simulink model "Cubli_2DOFv2"  (R2024b)
settings: Solver=FixedStepAuto  StartTime=0.0  StopTime=30  FixedStep=0.001  RelTol=1e-3  AbsTol=1e-3  EnableMultiTasking=on
values from neighbouring files (symbols this model uses):
  Km = 24.7*10^-3    (= 0.0247)    [cubli_2DOF_LQR.m]
  rad2rpm = 60/(2*pi)    (= 9.54929658551)    [cubli_2DOF_LQR.m]
  switch_time = 10    [cubli_2DOF_LQR.m]
undefined symbols (not defined in the file or in its folder): K, X, Y, Z
libraries: sm_lib x76, nesl_utility x8, simulink_extras x1
(part 2 of 3)

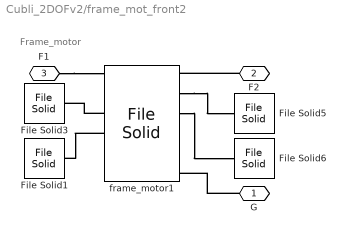
== system Cubli_2DOFv2/frame_mot_front2 ==
  note: Frame_motor
  File Solid{1,3,5..6} (4 alike) : sm_lib/Body Elements/File Solid  ExtGeomFileName=stp\socket countersunk head screw_iso.STEP  UnitType=FromFile  ExtGeomFileUnits=m  StepReaderType=HEX  ExportConvexHullGeometry=off  InertiaType=CalculateFromGeometry  BasedOnType=Mass  Density=1000  DensityUnits=kg/m^3  Mass=0.45  MassUnits=g  CenterOfMass=[0 0 0]  CenterOfMassUnits=m  MomentsOfInertia=[1 1 1]  MomentsOfInertiaUnits=kg*m^2  ProductsOfInertia=[0 0 0]  ProductsOfInertiaUnits=kg*m^2  GraphicType=FromGeometry  MarkerShape=Sphere  MarkerSize=10  GraphicVisPropType=SimpleVisualProperties  GraphicDiffuseColor=[0.502 0.502 0.502]  GraphicOpacity=1  GraphicSpecularColor=[0.5 0.5 0.5 1.0]  GraphicAmbientColor=[0.15 0.15 0.15 1.0]  GraphicEmissiveColor=[0.0 0.0 0.0 1.0]  GraphicShininess=75  DoExposeReferenceFrame=on  SerializedFrames=<Frames/>
  frame_motor1 : sm_lib/Body Elements/File Solid  ExtGeomFileName=stp\frame_motor.STEP  UnitType=FromFile  ExtGeomFileUnits=m  StepReaderType=HEX  ExportConvexHullGeometry=on  InertiaType=CalculateFromGeometry  BasedOnType=Mass  Density=1000  DensityUnits=kg/m^3  Mass=32  MassUnits=g  CenterOfMass=[0 0 0]  CenterOfMassUnits=m  MomentsOfInertia=[1 1 1]  MomentsOfInertiaUnits=kg*m^2  ProductsOfInertia=[0 0 0]  ProductsOfInertiaUnits=kg*m^2  GraphicType=FromGeometry  MarkerShape=Sphere  MarkerSize=10  GraphicVisPropType=SimpleVisualProperties  GraphicDiffuseColor=[0.902 0.902 0.902]  GraphicOpacity=1  GraphicSpecularColor=[0.5 0.5 0.5 1.0]  GraphicAmbientColor=[0.15 0.15 0.15 1.0]  GraphicEmissiveColor=[0.0 0.0 0.0 1.0]  GraphicShininess=75  DoExposeReferenceFrame=off  SerializedFrames=<Frames><Frame><Id>Frame1</Id><Value><Name>F1</Name><Origin><Source>GeometricFeature</Source><FeatureName>planar surface 14</FeatureName></Origin><PrimaryAxis><DefinedDirection>+Y</DefinedDirection><Source>ReferenceFrame</Source><SourceDirection>+Y</SourceDirection><FeatureName></FeatureName></PrimaryAxis><SecondaryAxis><DefinedDirection>+X</DefinedDirection><Source>ReferenceFrame</Source><SourceDirection>+X</SourceDirection><FeatureName></FeatureName></SecondaryAxis></Value></Frame><Frame><Id>Frame2</Id><Value><Name>F2</Name><Origin><Source>GeometricFeature</Source><FeatureName>planar surface 33</FeatureName></Origin><PrimaryAxis><DefinedDirection>+Z</DefinedDirection><Source>ReferenceFrame</Source><SourceDirection>+Z</SourceDirection><FeatureName></FeatureName></PrimaryAxis><SecondaryAxis><DefinedDirection>+X</DefinedDirection><Source>ReferenceFrame</Source><SourceDirection>+X</SourceDirection><FeatureName></FeatureName></SecondaryAxis></Value></Frame><Frame><Id>Frame3</Id><Value><Name>F3</Name><Origin><Source>GeometricFeature</Source><FeatureName>circular curve 13</FeatureName></Origin><PrimaryAxis><DefinedDirection>+Z</DefinedDirection><Source>ReferenceFrame</Source><SourceDirection>+Z</SourceDirection><FeatureName></FeatureName></PrimaryAxis><SecondaryAxis><DefinedDirection>+X</DefinedDirection><Source>ReferenceFrame</Source><SourceDirection>+X</SourceDirection><FeatureName></FeatureName></SecondaryAxis></Value></Frame><Frame><Id>Frame4</Id><Value><Name>F4</Name><Origin><Source>GeometricFeature</Source><FeatureName>circular curve 26</FeatureName></Origin><PrimaryAxis><DefinedDirection>+Y</DefinedDirection><Source>ReferenceFrame</Source><SourceDirection>+Y</SourceDirection><FeatureName></FeatureName></PrimaryAxis><SecondaryAxis><DefinedDirection>+X</DefinedDirection><Source>ReferenceFrame</Source><SourceDirection>-Z</SourceDirection><FeatureName></FeatureName></SecondaryAxis></Value></Frame><Frame><Id>Frame5</Id><Value><Name>F5</Name><Origin><Source>GeometricFeature</Source><FeatureName>circular curve 31</FeatureName></Origin><PrimaryAxis><DefinedDirection>+Y</DefinedDirection><Source>ReferenceFrame</Source><SourceDirection>+Y</SourceDirection><FeatureName></FeatureName></PrimaryAxis><SecondaryAxis><DefinedDirection>+X</DefinedDirection><Source>ReferenceFrame</Source><SourceDirection>-Z</SourceDirection><FeatureName></FeatureName></SecondaryAxis></Value></Frame><Frame><Id>Frame6</Id><Value><Name>F6</Name><Origin><Source>GeometricFeature</Source><FeatureName>circular curve 20</FeatureName></Origin><PrimaryAxis><DefinedDirection>+Y</DefinedDirection><Source>ReferenceFrame</Source><SourceDirection>+Y</SourceDirection><FeatureName></FeatureName></PrimaryAxis><SecondaryAxis><DefinedDirection>+X</DefinedDirection><Source>ReferenceFrame</Source><SourceDirection>-Z</SourceDirection><FeatureName></FeatureName></SecondaryAxis></Value></Frame><Frame><Id>Frame7</Id><Value><Name>F7</Name><Origin><Source>GeometricFeature</Source><FeatureName>circular curve 99</FeatureName></Origin><PrimaryAxis><DefinedDirection>+Y</DefinedDirection><Source>ReferenceFrame</Source><SourceDirection>+Y</SourceDirection><FeatureName></FeatureName></PrimaryAxis><SecondaryAxis><DefinedDirection>+X</DefinedDirection><Source>ReferenceFrame</Source><SourceDirection>-Z</SourceDirection><FeatureName></FeatureName></SecondaryAxis></Value></Frame><Frame><Id>Frame8</Id><Value><Name>F8</Name><Origin><Source>GeometricFeature</Source><FeatureName>circular curve 12</FeatureName></Origin><PrimaryAxis><DefinedDirection>+Y</DefinedDirection><Source>ReferenceFrame</Source><SourceDirection>+Y</SourceDirection><FeatureName></FeatureName></PrimaryAxis><SecondaryAxis><DefinedDirection>+X</DefinedDirection><Source>ReferenceFrame</Source><SourceDirection>-Z</SourceDirection><FeatureName></FeatureName></SecondaryAxis></Value></Frame><Frame><Id>Frame9</Id><Value><Name>F9</Name><Origin><Source>GeometricFeature</Source><FeatureName>circular curve 15</FeatureName></Origin><PrimaryAxis><DefinedDirection>+Y</DefinedDirection><Source>ReferenceFrame</Source><SourceDirection>+Y</SourceDirection><FeatureName></FeatureName></PrimaryAxis><SecondaryAxis><DefinedDirection>+X</DefinedDirection><Source>ReferenceFrame</Source><SourceDirection>-Z</SourceDirection><FeatureName></FeatureName></SecondaryAxis></Value></Frame><Frame><Id>Frame10</Id><Value><Name>F10</Name><Origin><Source>GeometricFeature</Source><FeatureName>circular curve 6</FeatureName></Origin><PrimaryAxis><DefinedDirection>+Y</DefinedDirection><Source>ReferenceFrame</Source><SourceDirection>+Y</SourceDirection><FeatureName></FeatureName></PrimaryAxis><SecondaryAxis><DefinedDirection>+X</DefinedDirection><Source>ReferenceFrame</Source><SourceDirection>-Z</SourceDirection><FeatureName></FeatureName></SecondaryAxis></Value></Frame><Frame><Id>Frame11</Id><Value><Name>F11</Name><Origin><Source>GeometricFeature</Source><FeatureName>circular curve 81</FeatureName></Origin><PrimaryAxis><DefinedDirection>+Y</DefinedDirection><Source>ReferenceFrame</Source><SourceDirection>+Y</SourceDirection><FeatureName></FeatureName></PrimaryAxis><SecondaryAxis><DefinedDirection>+X</DefinedDirection><Source>ReferenceFrame</Source><SourceDirection>-Z</SourceDirection><FeatureName></FeatureName></SecondaryAxis></Value></Frame></Frames>
  G : PMIOPort  Side=Left
  F2 : PMIOPort  Port=2  Side=Left
  F1 : PMIOPort  Port=3  Side=Right
  connections:
  G/RConn1 -- frame_motor1/RConn6
  F2/RConn1 -- frame_motor1/RConn1
  F1/RConn1 -- frame_motor1/LConn1
  frame_motor1/LConn4 -- File Solid1/RConn1
  frame_motor1/RConn3 -- File Solid6/RConn1
  frame_motor1/RConn2 -- File Solid5/RConn1
  frame_motor1/LConn3 -- File Solid3/RConn1

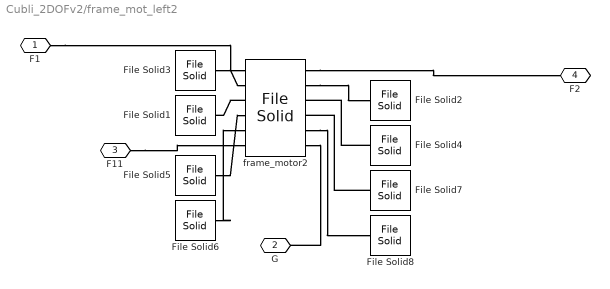
== system Cubli_2DOFv2/frame_mot_left2 ==
  File Solid{1..8} (8 alike) : sm_lib/Body Elements/File Solid  ExtGeomFileName=stp\socket countersunk head screw_iso.STEP  UnitType=FromFile  ExtGeomFileUnits=m  StepReaderType=HEX  ExportConvexHullGeometry=off  InertiaType=CalculateFromGeometry  BasedOnType=Mass  Density=1000  DensityUnits=kg/m^3  Mass=0.45  MassUnits=g  CenterOfMass=[0 0 0]  CenterOfMassUnits=m  MomentsOfInertia=[1 1 1]  MomentsOfInertiaUnits=kg*m^2  ProductsOfInertia=[0 0 0]  ProductsOfInertiaUnits=kg*m^2  GraphicType=FromGeometry  MarkerShape=Sphere  MarkerSize=10  GraphicVisPropType=SimpleVisualProperties  GraphicDiffuseColor=[0.502 0.502 0.502]  GraphicOpacity=1  GraphicSpecularColor=[0.5 0.5 0.5 1.0]  GraphicAmbientColor=[0.15 0.15 0.15 1.0]  GraphicEmissiveColor=[0.0 0.0 0.0 1.0]  GraphicShininess=75  DoExposeReferenceFrame=on  SerializedFrames=<Frames/>
  frame_motor2 : sm_lib/Body Elements/File Solid  ExtGeomFileName=stp\frame_motor.STEP  UnitType=FromFile  ExtGeomFileUnits=m  StepReaderType=HEX  ExportConvexHullGeometry=on  InertiaType=CalculateFromGeometry  BasedOnType=Mass  Density=1000  DensityUnits=kg/m^3  Mass=32  MassUnits=g  CenterOfMass=[0 0 0]  CenterOfMassUnits=m  MomentsOfInertia=[1 1 1]  MomentsOfInertiaUnits=kg*m^2  ProductsOfInertia=[0 0 0]  ProductsOfInertiaUnits=kg*m^2  GraphicType=FromGeometry  MarkerShape=Sphere  MarkerSize=10  GraphicVisPropType=SimpleVisualProperties  GraphicDiffuseColor=[0.902 0.902 0.902]  GraphicOpacity=1  GraphicSpecularColor=[0.5 0.5 0.5 1.0]  GraphicAmbientColor=[0.15 0.15 0.15 1.0]  GraphicEmissiveColor=[0.0 0.0 0.0 1.0]  GraphicShininess=75  DoExposeReferenceFrame=off  SerializedFrames=<Frames><Frame><Id>Frame1</Id><Value><Name>F1</Name><Origin><Source>GeometricFeature</Source><FeatureName>planar surface 33</FeatureName></Origin><PrimaryAxis><DefinedDirection>+X</DefinedDirection><Source>ReferenceFrame</Source><SourceDirection>+X</SourceDirection><FeatureName></FeatureName></PrimaryAxis><SecondaryAxis><DefinedDirection>+Y</DefinedDirection><Source>ReferenceFrame</Source><SourceDirection>-Y</SourceDirection><FeatureName></FeatureName></SecondaryAxis></Value></Frame><Frame><Id>Frame2</Id><Value><Name>F2</Name><Origin><Source>GeometricFeature</Source><FeatureName>planar surface 14</FeatureName></Origin><PrimaryAxis><DefinedDirection>+Z</DefinedDirection><Source>ReferenceFrame</Source><SourceDirection>+Z</SourceDirection><FeatureName></FeatureName></PrimaryAxis><SecondaryAxis><DefinedDirection>+X</DefinedDirection><Source>ReferenceFrame</Source><SourceDirection>+X</SourceDirection><FeatureName></FeatureName></SecondaryAxis></Value></Frame><Frame><Id>Frame3</Id><Value><Name>F3</Name><Origin><Source>GeometricFeature</Source><FeatureName>circular curve 26</FeatureName></Origin><PrimaryAxis><DefinedDirection>+Y</DefinedDirection><Source>ReferenceFrame</Source><SourceDirection>+Y</SourceDirection><FeatureName></FeatureName></PrimaryAxis><SecondaryAxis><DefinedDirection>+X</DefinedDirection><Source>ReferenceFrame</Source><SourceDirection>-Z</SourceDirection><FeatureName></FeatureName></SecondaryAxis></Value></Frame><Frame><Id>Frame4</Id><Value><Name>F4</Name><Origin><Source>GeometricFeature</Source><FeatureName>circular curve 118</FeatureName></Origin><PrimaryAxis><DefinedDirection>+Y</DefinedDirection><Source>ReferenceFrame</Source><SourceDirection>+Y</SourceDirection><FeatureName></FeatureName></PrimaryAxis><SecondaryAxis><DefinedDirection>+X</DefinedDirection><Source>ReferenceFrame</Source><SourceDirection>-Z</SourceDirection><FeatureName></FeatureName></SecondaryAxis></Value></Frame><Frame><Id>Frame5</Id><Value><Name>F5</Name><Origin><Source>GeometricFeature</Source><FeatureName>circular curve 20</FeatureName></Origin><PrimaryAxis><DefinedDirection>+Y</DefinedDirection><Source>ReferenceFrame</Source><SourceDirection>+Y</SourceDirection><FeatureName></FeatureName></PrimaryAxis><SecondaryAxis><DefinedDirection>+X</DefinedDirection><Source>ReferenceFrame</Source><SourceDirection>-Z</SourceDirection><FeatureName></FeatureName></SecondaryAxis></Value></Frame><Frame><Id>Frame6</Id><Value><Name>F6</Name><Origin><Source>GeometricFeature</Source><FeatureName>circular curve 99</FeatureName></Origin><PrimaryAxis><DefinedDirection>+Y</DefinedDirection><Source>ReferenceFrame</Source><SourceDirection>+Y</SourceDirection><FeatureName></FeatureName></PrimaryAxis><SecondaryAxis><DefinedDirection>+X</DefinedDirection><Source>ReferenceFrame</Source><SourceDirection>-Z</SourceDirection><FeatureName></FeatureName></SecondaryAxis></Value></Frame><Frame><Id>Frame7</Id><Value><Name>F7</Name><Origin><Source>GeometricFeature</Source><FeatureName>circular curve 6</FeatureName></Origin><PrimaryAxis><DefinedDirection>+Y</DefinedDirection><Source>ReferenceFrame</Source><SourceDirection>+Y</SourceDirection><FeatureName></FeatureName></PrimaryAxis><SecondaryAxis><DefinedDirection>+X</DefinedDirection><Source>ReferenceFrame</Source><SourceDirection>-Z</SourceDirection><FeatureName></FeatureName></SecondaryAxis></Value></Frame><Frame><Id>Frame8</Id><Value><Name>F8</Name><Origin><Source>GeometricFeature</Source><FeatureName>circular curve 92</FeatureName></Origin><PrimaryAxis><DefinedDirection>+Y</DefinedDirection><Source>ReferenceFrame</Source><SourceDirection>+Y</SourceDirection><FeatureName></FeatureName></PrimaryAxis><SecondaryAxis><DefinedDirection>+X</DefinedDirection><Source>ReferenceFrame</Source><SourceDirection>-Z</SourceDirection><FeatureName></FeatureName></SecondaryAxis></Value></Frame><Frame><Id>Frame9</Id><Value><Name>F9</Name><Origin><Source>GeometricFeature</Source><FeatureName>circular curve 15</FeatureName></Origin><PrimaryAxis><DefinedDirection>+Y</DefinedDirection><Source>ReferenceFrame</Source><SourceDirection>+Y</SourceDirection><FeatureName></FeatureName></PrimaryAxis><SecondaryAxis><DefinedDirection>+X</DefinedDirection><Source>ReferenceFrame</Source><SourceDirection>-Z</SourceDirection><FeatureName></FeatureName></SecondaryAxis></Value></Frame><Frame><Id>Frame10</Id><Value><Name>F10</Name><Origin><Source>GeometricFeature</Source><FeatureName>circular curve 81</FeatureName></Origin><PrimaryAxis><DefinedDirection>+Y</DefinedDirection><Source>ReferenceFrame</Source><SourceDirection>+Y</SourceDirection><FeatureName></FeatureName></PrimaryAxis><SecondaryAxis><DefinedDirection>+X</DefinedDirection><Source>ReferenceFrame</Source><SourceDirection>-Z</SourceDirection><FeatureName></FeatureName></SecondaryAxis></Value></Frame><Frame><Id>Frame11</Id><Value><Name>F11</Name><Origin><Source>GeometricFeature</Source><FeatureName>circular curve 68</FeatureName></Origin><PrimaryAxis><DefinedDirection>+Z</DefinedDirection><Source>ReferenceFrame</Source><SourceDirection>+Z</SourceDirection><FeatureName></FeatureName></PrimaryAxis><SecondaryAxis><DefinedDirection>+X</DefinedDirection><Source>ReferenceFrame</Source><SourceDirection>+X</SourceDirection><FeatureName></FeatureName></SecondaryAxis></Value></Frame></Frames>
  F1 : PMIOPort  Side=Left
  G : PMIOPort  Port=2  Side=Left
  F11 : PMIOPort  Port=3  Side=Right
  F2 : PMIOPort  Port=4  Side=Right
  connections:
  F11/RConn1 -- frame_motor2/LConn6
  frame_motor2/RConn5 -- File Solid8/RConn1
  File Solid7/RConn1 -- frame_motor2/RConn4
  File Solid6/RConn1 -- frame_motor2/LConn5
  File Solid5/RConn1 -- frame_motor2/LConn4
  frame_motor2/RConn6 -- G/RConn1
  F1/RConn1 -- frame_motor2/LConn1
  File Solid4/RConn1 -- frame_motor2/RConn3
  frame_motor2/RConn2 -- File Solid2/RConn1
  frame_motor2/RConn1 -- F2/RConn1
  frame_motor2/LConn3 -- File Solid1/RConn1
  File Solid3/RConn1 -- frame_motor2/LConn2

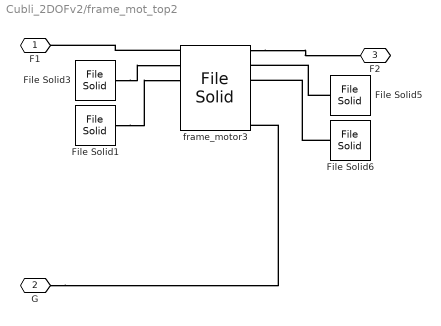
== system Cubli_2DOFv2/frame_mot_top2 ==
  File Solid{1,3,5..6} (4 alike) : sm_lib/Body Elements/File Solid  ExtGeomFileName=stp\socket countersunk head screw_iso.STEP  UnitType=FromFile  ExtGeomFileUnits=m  StepReaderType=HEX  ExportConvexHullGeometry=off  InertiaType=CalculateFromGeometry  BasedOnType=Mass  Density=1000  DensityUnits=kg/m^3  Mass=0.45  MassUnits=g  CenterOfMass=[0 0 0]  CenterOfMassUnits=m  MomentsOfInertia=[1 1 1]  MomentsOfInertiaUnits=kg*m^2  ProductsOfInertia=[0 0 0]  ProductsOfInertiaUnits=kg*m^2  GraphicType=FromGeometry  MarkerShape=Sphere  MarkerSize=10  GraphicVisPropType=SimpleVisualProperties  GraphicDiffuseColor=[0.502 0.502 0.502]  GraphicOpacity=1  GraphicSpecularColor=[0.5 0.5 0.5 1.0]  GraphicAmbientColor=[0.15 0.15 0.15 1.0]  GraphicEmissiveColor=[0.0 0.0 0.0 1.0]  GraphicShininess=75  DoExposeReferenceFrame=on  SerializedFrames=<Frames/>
  frame_motor3 : sm_lib/Body Elements/File Solid  ExtGeomFileName=stp\frame_motor.STEP  UnitType=FromFile  ExtGeomFileUnits=m  StepReaderType=HEX  ExportConvexHullGeometry=on  InertiaType=CalculateFromGeometry  BasedOnType=Mass  Density=1000  DensityUnits=kg/m^3  Mass=32  MassUnits=g  CenterOfMass=[0 0 0]  CenterOfMassUnits=m  MomentsOfInertia=[1 1 1]  MomentsOfInertiaUnits=kg*m^2  ProductsOfInertia=[0 0 0]  ProductsOfInertiaUnits=kg*m^2  GraphicType=FromGeometry  MarkerShape=Sphere  MarkerSize=10  GraphicVisPropType=SimpleVisualProperties  GraphicDiffuseColor=[0.902 0.902 0.902]  GraphicOpacity=1  GraphicSpecularColor=[0.5 0.5 0.5 1.0]  GraphicAmbientColor=[0.15 0.15 0.15 1.0]  GraphicEmissiveColor=[0.0 0.0 0.0 1.0]  GraphicShininess=75  DoExposeReferenceFrame=off  SerializedFrames=<Frames><Frame><Id>Frame1</Id><Value><Name>F1</Name><Origin><Source>GeometricFeature</Source><FeatureName>planar surface 33</FeatureName></Origin><PrimaryAxis><DefinedDirection>+Z</DefinedDirection><Source>ReferenceFrame</Source><SourceDirection>+Z</SourceDirection><FeatureName></FeatureName></PrimaryAxis><SecondaryAxis><DefinedDirection>+X</DefinedDirection><Source>ReferenceFrame</Source><SourceDirection>+X</SourceDirection><FeatureName></FeatureName></SecondaryAxis></Value></Frame><Frame><Id>Frame2</Id><Value><Name>F2</Name><Origin><Source>GeometricFeature</Source><FeatureName>planar surface 14</FeatureName></Origin><PrimaryAxis><DefinedDirection>+Z</DefinedDirection><Source>ReferenceFrame</Source><SourceDirection>+Z</SourceDirection><FeatureName></FeatureName></PrimaryAxis><SecondaryAxis><DefinedDirection>+X</DefinedDirection><Source>ReferenceFrame</Source><SourceDirection>+X</SourceDirection><FeatureName></FeatureName></SecondaryAxis></Value></Frame><Frame><Id>Frame3</Id><Value><Name>F3</Name><Origin><Source>GeometricFeature</Source><FeatureName>circular curve 26</FeatureName></Origin><PrimaryAxis><DefinedDirection>+Y</DefinedDirection><Source>ReferenceFrame</Source><SourceDirection>+Y</SourceDirection><FeatureName></FeatureName></PrimaryAxis><SecondaryAxis><DefinedDirection>+X</DefinedDirection><Source>ReferenceFrame</Source><SourceDirection>-Z</SourceDirection><FeatureName></FeatureName></SecondaryAxis></Value></Frame><Frame><Id>Frame4</Id><Value><Name>F4</Name><Origin><Source>GeometricFeature</Source><FeatureName>circular curve 31</FeatureName></Origin><PrimaryAxis><DefinedDirection>+Y</DefinedDirection><Source>ReferenceFrame</Source><SourceDirection>+Y</SourceDirection><FeatureName></FeatureName></PrimaryAxis><SecondaryAxis><DefinedDirection>+X</DefinedDirection><Source>ReferenceFrame</Source><SourceDirection>-Z</SourceDirection><FeatureName></FeatureName></SecondaryAxis></Value></Frame><Frame><Id>Frame5</Id><Value><Name>F5</Name><Origin><Source>GeometricFeature</Source><FeatureName>circular curve 20</FeatureName></Origin><PrimaryAxis><DefinedDirection>+Y</DefinedDirection><Source>ReferenceFrame</Source><SourceDirection>+Y</SourceDirection><FeatureName></FeatureName></PrimaryAxis><SecondaryAxis><DefinedDirection>+X</DefinedDirection><Source>ReferenceFrame</Source><SourceDirection>-Z</SourceDirection><FeatureName></FeatureName></SecondaryAxis></Value></Frame><Frame><Id>Frame6</Id><Value><Name>F6</Name><Origin><Source>GeometricFeature</Source><FeatureName>circular curve 23</FeatureName></Origin><PrimaryAxis><DefinedDirection>+Y</DefinedDirection><Source>ReferenceFrame</Source><SourceDirection>+Y</SourceDirection><FeatureName></FeatureName></PrimaryAxis><SecondaryAxis><DefinedDirection>+X</DefinedDirection><Source>ReferenceFrame</Source><SourceDirection>-Z</SourceDirection><FeatureName></FeatureName></SecondaryAxis></Value></Frame><Frame><Id>Frame7</Id><Value><Name>F7</Name><Origin><Source>GeometricFeature</Source><FeatureName>circular curve 6</FeatureName></Origin><PrimaryAxis><DefinedDirection>+Y</DefinedDirection><Source>ReferenceFrame</Source><SourceDirection>+Y</SourceDirection><FeatureName></FeatureName></PrimaryAxis><SecondaryAxis><DefinedDirection>+X</DefinedDirection><Source>ReferenceFrame</Source><SourceDirection>-Z</SourceDirection><FeatureName></FeatureName></SecondaryAxis></Value></Frame><Frame><Id>Frame8</Id><Value><Name>F8</Name><Origin><Source>GeometricFeature</Source><FeatureName>circular curve 92</FeatureName></Origin><PrimaryAxis><DefinedDirection>+Y</DefinedDirection><Source>ReferenceFrame</Source><SourceDirection>+Y</SourceDirection><FeatureName></FeatureName></PrimaryAxis><SecondaryAxis><DefinedDirection>+X</DefinedDirection><Source>ReferenceFrame</Source><SourceDirection>-Z</SourceDirection><FeatureName></FeatureName></SecondaryAxis></Value></Frame><Frame><Id>Frame9</Id><Value><Name>F9</Name><Origin><Source>GeometricFeature</Source><FeatureName>circular curve 93</FeatureName></Origin><PrimaryAxis><DefinedDirection>+Y</DefinedDirection><Source>ReferenceFrame</Source><SourceDirection>+Y</SourceDirection><FeatureName></FeatureName></PrimaryAxis><SecondaryAxis><DefinedDirection>+X</DefinedDirection><Source>ReferenceFrame</Source><SourceDirection>-Z</SourceDirection><FeatureName></FeatureName></SecondaryAxis></Value></Frame><Frame><Id>Frame10</Id><Value><Name>F10</Name><Origin><Source>GeometricFeature</Source><FeatureName>circular curve 81</FeatureName></Origin><PrimaryAxis><DefinedDirection>+Y</DefinedDirection><Source>ReferenceFrame</Source><SourceDirection>+Y</SourceDirection><FeatureName></FeatureName></PrimaryAxis><SecondaryAxis><DefinedDirection>+X</DefinedDirection><Source>ReferenceFrame</Source><SourceDirection>-Z</SourceDirection><FeatureName></FeatureName></SecondaryAxis></Value></Frame><Frame><Id>Frame11</Id><Value><Name>F11</Name><Origin><Source>GeometricFeature</Source><FeatureName>circular curve 68</FeatureName></Origin><PrimaryAxis><DefinedDirection>+Z</DefinedDirection><Source>ReferenceFrame</Source><SourceDirection>+Z</SourceDirection><FeatureName></FeatureName></PrimaryAxis><SecondaryAxis><DefinedDirection>+X</DefinedDirection><Source>ReferenceFrame</Source><SourceDirection>+X</SourceDirection><FeatureName></FeatureName></SecondaryAxis></Value></Frame></Frames>
  F1 : PMIOPort  Side=Left
  G : PMIOPort  Port=2  Side=Left
  F2 : PMIOPort  Port=3  Side=Right
  connections:
  frame_motor3/LConn1 -- F1/RConn1
  File Solid5/RConn1 -- frame_motor3/RConn2
  File Solid1/RConn1 -- frame_motor3/LConn3
  frame_motor3/RConn1 -- F2/RConn1
  File Solid3/RConn1 -- frame_motor3/LConn2
  G/RConn1 -- frame_motor3/RConn6
  File Solid6/RConn1 -- frame_motor3/RConn3

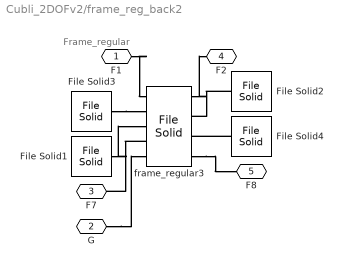
== system Cubli_2DOFv2/frame_reg_back2 ==
  note: Frame_regular
  File Solid{1..4} (4 alike) : sm_lib/Body Elements/File Solid  ExtGeomFileName=stp\socket countersunk head screw_iso.STEP  UnitType=FromFile  ExtGeomFileUnits=m  StepReaderType=HEX  ExportConvexHullGeometry=off  InertiaType=CalculateFromGeometry  BasedOnType=Mass  Density=1000  DensityUnits=kg/m^3  Mass=0.45  MassUnits=g  CenterOfMass=[0 0 0]  CenterOfMassUnits=m  MomentsOfInertia=[1 1 1]  MomentsOfInertiaUnits=kg*m^2  ProductsOfInertia=[0 0 0]  ProductsOfInertiaUnits=kg*m^2  GraphicType=FromGeometry  MarkerShape=Sphere  MarkerSize=10  GraphicVisPropType=SimpleVisualProperties  GraphicDiffuseColor=[0.502 0.502 0.502]  GraphicOpacity=1  GraphicSpecularColor=[0.5 0.5 0.5 1.0]  GraphicAmbientColor=[0.15 0.15 0.15 1.0]  GraphicEmissiveColor=[0.0 0.0 0.0 1.0]  GraphicShininess=75  DoExposeReferenceFrame=on  SerializedFrames=<Frames/>
  frame_regular3 : sm_lib/Body Elements/File Solid  ExtGeomFileName=stp\frame_regular.STEP  UnitType=FromFile  ExtGeomFileUnits=m  StepReaderType=HEX  ExportConvexHullGeometry=on  InertiaType=CalculateFromGeometry  BasedOnType=Mass  Density=1000  DensityUnits=kg/m^3  Mass=27  MassUnits=g  CenterOfMass=[0 0 0]  CenterOfMassUnits=m  MomentsOfInertia=[1 1 1]  MomentsOfInertiaUnits=kg*m^2  ProductsOfInertia=[0 0 0]  ProductsOfInertiaUnits=kg*m^2  GraphicType=FromGeometry  MarkerShape=Sphere  MarkerSize=10  GraphicVisPropType=SimpleVisualProperties  GraphicDiffuseColor=[0.902 0.902 0.902]  GraphicOpacity=1  GraphicSpecularColor=[0.5 0.5 0.5 1.0]  GraphicAmbientColor=[0.15 0.15 0.15 1.0]  GraphicEmissiveColor=[0.0 0.0 0.0 1.0]  GraphicShininess=75  DoExposeReferenceFrame=off  SerializedFrames=<Frames><Frame><Id>Frame1</Id><Value><Name>F1</Name><Origin><Source>GeometricFeature</Source><FeatureName>planar surface 10</FeatureName></Origin><PrimaryAxis><DefinedDirection>+Y</DefinedDirection><Source>ReferenceFrame</Source><SourceDirection>-Z</SourceDirection><FeatureName></FeatureName></PrimaryAxis><SecondaryAxis><DefinedDirection>+Z</DefinedDirection><Source>ReferenceFrame</Source><SourceDirection>-X</SourceDirection><FeatureName></FeatureName></SecondaryAxis></Value></Frame><Frame><Id>Frame2</Id><Value><Name>F2</Name><Origin><Source>GeometricFeature</Source><FeatureName>planar surface 19</FeatureName></Origin><PrimaryAxis><DefinedDirection>+Z</DefinedDirection><Source>ReferenceFrame</Source><SourceDirection>+Z</SourceDirection><FeatureName></FeatureName></PrimaryAxis><SecondaryAxis><DefinedDirection>+X</DefinedDirection><Source>ReferenceFrame</Source><SourceDirection>+X</SourceDirection><FeatureName></FeatureName></SecondaryAxis></Value></Frame><Frame><Id>Frame3</Id><Value><Name>F3</Name><Origin><Source>GeometricFeature</Source><FeatureName>circular curve 65</FeatureName></Origin><PrimaryAxis><DefinedDirection>+Y</DefinedDirection><Source>ReferenceFrame</Source><SourceDirection>+Y</SourceDirection><FeatureName></FeatureName></PrimaryAxis><SecondaryAxis><DefinedDirection>+X</DefinedDirection><Source>ReferenceFrame</Source><SourceDirection>-Z</SourceDirection><FeatureName></FeatureName></SecondaryAxis></Value></Frame><Frame><Id>Frame4</Id><Value><Name>F4</Name><Origin><Source>GeometricFeature</Source><FeatureName>circular curve 64</FeatureName></Origin><PrimaryAxis><DefinedDirection>+Y</DefinedDirection><Source>ReferenceFrame</Source><SourceDirection>+Y</SourceDirection><FeatureName></FeatureName></PrimaryAxis><SecondaryAxis><DefinedDirection>+X</DefinedDirection><Source>ReferenceFrame</Source><SourceDirection>-Z</SourceDirection><FeatureName></FeatureName></SecondaryAxis></Value></Frame><Frame><Id>Frame5</Id><Value><Name>F5</Name><Origin><Source>GeometricFeature</Source><FeatureName>circular curve 7</FeatureName></Origin><PrimaryAxis><DefinedDirection>+Y</DefinedDirection><Source>ReferenceFrame</Source><SourceDirection>+Y</SourceDirection><FeatureName></FeatureName></PrimaryAxis><SecondaryAxis><DefinedDirection>+X</DefinedDirection><Source>ReferenceFrame</Source><SourceDirection>-Z</SourceDirection><FeatureName></FeatureName></SecondaryAxis></Value></Frame><Frame><Id>Frame6</Id><Value><Name>F6</Name><Origin><Source>GeometricFeature</Source><FeatureName>circular curve 17</FeatureName></Origin><PrimaryAxis><DefinedDirection>+Y</DefinedDirection><Source>ReferenceFrame</Source><SourceDirection>+Y</SourceDirection><FeatureName></FeatureName></PrimaryAxis><SecondaryAxis><DefinedDirection>+X</DefinedDirection><Source>ReferenceFrame</Source><SourceDirection>-Z</SourceDirection><FeatureName></FeatureName></SecondaryAxis></Value></Frame><Frame><Id>Frame7</Id><Value><Name>F7</Name><Origin><Source>GeometricFeature</Source><FeatureName>planar surface 21</FeatureName></Origin><PrimaryAxis><DefinedDirection>+Z</DefinedDirection><Source>ReferenceFrame</Source><SourceDirection>+Z</SourceDirection><FeatureName></FeatureName></PrimaryAxis><SecondaryAxis><DefinedDirection>+X</DefinedDirection><Source>ReferenceFrame</Source><SourceDirection>+X</SourceDirection><FeatureName></FeatureName></SecondaryAxis></Value></Frame><Frame><Id>Frame8</Id><Value><Name>F8</Name><Origin><Source>GeometricFeature</Source><FeatureName>circular curve 5</FeatureName></Origin><PrimaryAxis><DefinedDirection>+Z</DefinedDirection><Source>ReferenceFrame</Source><SourceDirection>+Z</SourceDirection><FeatureName></FeatureName></PrimaryAxis><SecondaryAxis><DefinedDirection>+X</DefinedDirection><Source>ReferenceFrame</Source><SourceDirection>+X</SourceDirection><FeatureName></FeatureName></SecondaryAxis></Value></Frame></Frames>
  F1 : PMIOPort  Side=Left
  G : PMIOPort  Port=2  Side=Left
  F7 : PMIOPort  Port=3  Side=Left
  F2 : PMIOPort  Port=4  Side=Right
  F8 : PMIOPort  Port=5  Side=Right
  connections:
  frame_regular3/RConn1 -- F2/RConn1
  F1/RConn1 -- frame_regular3/LConn1
  File Solid3/RConn1 -- frame_regular3/LConn2
  File Solid1/RConn1 -- frame_regular3/LConn3
  File Solid4/RConn1 -- frame_regular3/RConn3
  File Solid2/RConn1 -- frame_regular3/RConn2
  frame_regular3/LConn4 -- F7/RConn1
  G/RConn1 -- frame_regular3/LConn5
  frame_regular3/RConn4 -- F8/RConn1

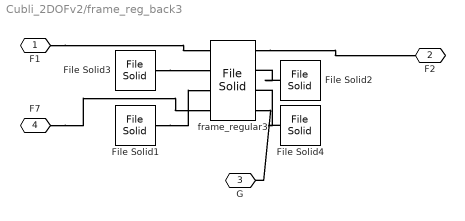
== system Cubli_2DOFv2/frame_reg_back3 ==
  File Solid{1..4} (4 alike) : sm_lib/Body Elements/File Solid  ExtGeomFileName=stp\socket countersunk head screw_iso.STEP  UnitType=FromFile  ExtGeomFileUnits=m  StepReaderType=HEX  ExportConvexHullGeometry=off  InertiaType=CalculateFromGeometry  BasedOnType=Mass  Density=1000  DensityUnits=kg/m^3  Mass=0.45  MassUnits=g  CenterOfMass=[0 0 0]  CenterOfMassUnits=m  MomentsOfInertia=[1 1 1]  MomentsOfInertiaUnits=kg*m^2  ProductsOfInertia=[0 0 0]  ProductsOfInertiaUnits=kg*m^2  GraphicType=FromGeometry  MarkerShape=Sphere  MarkerSize=10  GraphicVisPropType=SimpleVisualProperties  GraphicDiffuseColor=[0.502 0.502 0.502]  GraphicOpacity=1  GraphicSpecularColor=[0.5 0.5 0.5 1.0]  GraphicAmbientColor=[0.15 0.15 0.15 1.0]  GraphicEmissiveColor=[0.0 0.0 0.0 1.0]  GraphicShininess=75  DoExposeReferenceFrame=on  SerializedFrames=<Frames/>
  frame_regular3 : sm_lib/Body Elements/File Solid  ExtGeomFileName=stp\frame_regular.STEP  UnitType=FromFile  ExtGeomFileUnits=m  StepReaderType=HEX  ExportConvexHullGeometry=on  InertiaType=CalculateFromGeometry  BasedOnType=Mass  Density=1000  DensityUnits=kg/m^3  Mass=27  MassUnits=g  CenterOfMass=[0 0 0]  CenterOfMassUnits=m  MomentsOfInertia=[1 1 1]  MomentsOfInertiaUnits=kg*m^2  ProductsOfInertia=[0 0 0]  ProductsOfInertiaUnits=kg*m^2  GraphicType=FromGeometry  MarkerShape=Sphere  MarkerSize=10  GraphicVisPropType=SimpleVisualProperties  GraphicDiffuseColor=[0.902 0.902 0.902]  GraphicOpacity=1  GraphicSpecularColor=[0.5 0.5 0.5 1.0]  GraphicAmbientColor=[0.15 0.15 0.15 1.0]  GraphicEmissiveColor=[0.0 0.0 0.0 1.0]  GraphicShininess=75  DoExposeReferenceFrame=off  SerializedFrames=<Frames><Frame><Id>Frame1</Id><Value><Name>F1</Name><Origin><Source>GeometricFeature</Source><FeatureName>planar surface 10</FeatureName></Origin><PrimaryAxis><DefinedDirection>+Y</DefinedDirection><Source>ReferenceFrame</Source><SourceDirection>-Z</SourceDirection><FeatureName></FeatureName></PrimaryAxis><SecondaryAxis><DefinedDirection>+Z</DefinedDirection><Source>ReferenceFrame</Source><SourceDirection>-X</SourceDirection><FeatureName></FeatureName></SecondaryAxis></Value></Frame><Frame><Id>Frame2</Id><Value><Name>F2</Name><Origin><Source>GeometricFeature</Source><FeatureName>planar surface 19</FeatureName></Origin><PrimaryAxis><DefinedDirection>+Z</DefinedDirection><Source>ReferenceFrame</Source><SourceDirection>+Z</SourceDirection><FeatureName></FeatureName></PrimaryAxis><SecondaryAxis><DefinedDirection>+X</DefinedDirection><Source>ReferenceFrame</Source><SourceDirection>+X</SourceDirection><FeatureName></FeatureName></SecondaryAxis></Value></Frame><Frame><Id>Frame3</Id><Value><Name>F3</Name><Origin><Source>GeometricFeature</Source><FeatureName>circular curve 65</FeatureName></Origin><PrimaryAxis><DefinedDirection>+Y</DefinedDirection><Source>ReferenceFrame</Source><SourceDirection>+Y</SourceDirection><FeatureName></FeatureName></PrimaryAxis><SecondaryAxis><DefinedDirection>+X</DefinedDirection><Source>ReferenceFrame</Source><SourceDirection>-Z</SourceDirection><FeatureName></FeatureName></SecondaryAxis></Value></Frame><Frame><Id>Frame4</Id><Value><Name>F4</Name><Origin><Source>GeometricFeature</Source><FeatureName>circular curve 64</FeatureName></Origin><PrimaryAxis><DefinedDirection>+Y</DefinedDirection><Source>ReferenceFrame</Source><SourceDirection>+Y</SourceDirection><FeatureName></FeatureName></PrimaryAxis><SecondaryAxis><DefinedDirection>+X</DefinedDirection><Source>ReferenceFrame</Source><SourceDirection>-Z</SourceDirection><FeatureName></FeatureName></SecondaryAxis></Value></Frame><Frame><Id>Frame5</Id><Value><Name>F5</Name><Origin><Source>GeometricFeature</Source><FeatureName>circular curve 7</FeatureName></Origin><PrimaryAxis><DefinedDirection>+Y</DefinedDirection><Source>ReferenceFrame</Source><SourceDirection>+Y</SourceDirection><FeatureName></FeatureName></PrimaryAxis><SecondaryAxis><DefinedDirection>+X</DefinedDirection><Source>ReferenceFrame</Source><SourceDirection>-Z</SourceDirection><FeatureName></FeatureName></SecondaryAxis></Value></Frame><Frame><Id>Frame6</Id><Value><Name>F6</Name><Origin><Source>GeometricFeature</Source><FeatureName>circular curve 17</FeatureName></Origin><PrimaryAxis><DefinedDirection>+Y</DefinedDirection><Source>ReferenceFrame</Source><SourceDirection>+Y</SourceDirection><FeatureName></FeatureName></PrimaryAxis><SecondaryAxis><DefinedDirection>+X</DefinedDirection><Source>ReferenceFrame</Source><SourceDirection>-Z</SourceDirection><FeatureName></FeatureName></SecondaryAxis></Value></Frame><Frame><Id>Frame7</Id><Value><Name>F7</Name><Origin><Source>GeometricFeature</Source><FeatureName>circular curve 120</FeatureName></Origin><PrimaryAxis><DefinedDirection>+Z</DefinedDirection><Source>ReferenceFrame</Source><SourceDirection>+Z</SourceDirection><FeatureName></FeatureName></PrimaryAxis><SecondaryAxis><DefinedDirection>+X</DefinedDirection><Source>ReferenceFrame</Source><SourceDirection>+X</SourceDirection><FeatureName></FeatureName></SecondaryAxis></Value></Frame></Frames>
  F1 : PMIOPort  Side=Left
  F2 : PMIOPort  Port=2  Side=Right
  G : PMIOPort  Port=3  Side=Left
  F7 : PMIOPort  Port=4  Side=Right
  connections:
  File Solid2/RConn1 -- frame_regular3/RConn2
  File Solid4/RConn1 -- frame_regular3/RConn3
  File Solid1/RConn1 -- frame_regular3/LConn3
  File Solid3/RConn1 -- frame_regular3/LConn2
  F1/RConn1 -- frame_regular3/LConn1
  frame_regular3/RConn1 -- F2/RConn1
  frame_regular3/RConn4 -- G/RConn1
  F7/RConn1 -- frame_regular3/LConn4

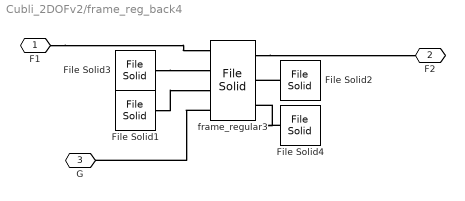
== system Cubli_2DOFv2/frame_reg_back4 ==
  File Solid{1..4} (4 alike) : sm_lib/Body Elements/File Solid  ExtGeomFileName=stp\socket countersunk head screw_iso.STEP  UnitType=FromFile  ExtGeomFileUnits=m  StepReaderType=HEX  ExportConvexHullGeometry=off  InertiaType=CalculateFromGeometry  BasedOnType=Mass  Density=1000  DensityUnits=kg/m^3  Mass=0.45  MassUnits=g  CenterOfMass=[0 0 0]  CenterOfMassUnits=m  MomentsOfInertia=[1 1 1]  MomentsOfInertiaUnits=kg*m^2  ProductsOfInertia=[0 0 0]  ProductsOfInertiaUnits=kg*m^2  GraphicType=FromGeometry  MarkerShape=Sphere  MarkerSize=10  GraphicVisPropType=SimpleVisualProperties  GraphicDiffuseColor=[0.502 0.502 0.502]  GraphicOpacity=1  GraphicSpecularColor=[0.5 0.5 0.5 1.0]  GraphicAmbientColor=[0.15 0.15 0.15 1.0]  GraphicEmissiveColor=[0.0 0.0 0.0 1.0]  GraphicShininess=75  DoExposeReferenceFrame=on  SerializedFrames=<Frames/>
  frame_regular3 : sm_lib/Body Elements/File Solid  ExtGeomFileName=stp\frame_regular.STEP  UnitType=FromFile  ExtGeomFileUnits=m  StepReaderType=HEX  ExportConvexHullGeometry=on  InertiaType=CalculateFromGeometry  BasedOnType=Mass  Density=1000  DensityUnits=kg/m^3  Mass=27  MassUnits=g  CenterOfMass=[0 0 0]  CenterOfMassUnits=m  MomentsOfInertia=[1 1 1]  MomentsOfInertiaUnits=kg*m^2  ProductsOfInertia=[0 0 0]  ProductsOfInertiaUnits=kg*m^2  GraphicType=FromGeometry  MarkerShape=Sphere  MarkerSize=10  GraphicVisPropType=SimpleVisualProperties  GraphicDiffuseColor=[0.902 0.902 0.902]  GraphicOpacity=1  GraphicSpecularColor=[0.5 0.5 0.5 1.0]  GraphicAmbientColor=[0.15 0.15 0.15 1.0]  GraphicEmissiveColor=[0.0 0.0 0.0 1.0]  GraphicShininess=75  DoExposeReferenceFrame=off  SerializedFrames=<Frames><Frame><Id>Frame1</Id><Value><Name>F1</Name><Origin><Source>GeometricFeature</Source><FeatureName>planar surface 10</FeatureName></Origin><PrimaryAxis><DefinedDirection>+Y</DefinedDirection><Source>ReferenceFrame</Source><SourceDirection>-Z</SourceDirection><FeatureName></FeatureName></PrimaryAxis><SecondaryAxis><DefinedDirection>+Z</DefinedDirection><Source>ReferenceFrame</Source><SourceDirection>-X</SourceDirection><FeatureName></FeatureName></SecondaryAxis></Value></Frame><Frame><Id>Frame2</Id><Value><Name>F2</Name><Origin><Source>GeometricFeature</Source><FeatureName>planar surface 19</FeatureName></Origin><PrimaryAxis><DefinedDirection>+Z</DefinedDirection><Source>ReferenceFrame</Source><SourceDirection>+Z</SourceDirection><FeatureName></FeatureName></PrimaryAxis><SecondaryAxis><DefinedDirection>+X</DefinedDirection><Source>ReferenceFrame</Source><SourceDirection>+X</SourceDirection><FeatureName></FeatureName></SecondaryAxis></Value></Frame><Frame><Id>Frame3</Id><Value><Name>F3</Name><Origin><Source>GeometricFeature</Source><FeatureName>circular curve 65</FeatureName></Origin><PrimaryAxis><DefinedDirection>+Y</DefinedDirection><Source>ReferenceFrame</Source><SourceDirection>+Y</SourceDirection><FeatureName></FeatureName></PrimaryAxis><SecondaryAxis><DefinedDirection>+X</DefinedDirection><Source>ReferenceFrame</Source><SourceDirection>-Z</SourceDirection><FeatureName></FeatureName></SecondaryAxis></Value></Frame><Frame><Id>Frame4</Id><Value><Name>F4</Name><Origin><Source>GeometricFeature</Source><FeatureName>circular curve 64</FeatureName></Origin><PrimaryAxis><DefinedDirection>+Y</DefinedDirection><Source>ReferenceFrame</Source><SourceDirection>+Y</SourceDirection><FeatureName></FeatureName></PrimaryAxis><SecondaryAxis><DefinedDirection>+X</DefinedDirection><Source>ReferenceFrame</Source><SourceDirection>-Z</SourceDirection><FeatureName></FeatureName></SecondaryAxis></Value></Frame><Frame><Id>Frame5</Id><Value><Name>F5</Name><Origin><Source>GeometricFeature</Source><FeatureName>circular curve 7</FeatureName></Origin><PrimaryAxis><DefinedDirection>+Y</DefinedDirection><Source>ReferenceFrame</Source><SourceDirection>+Y</SourceDirection><FeatureName></FeatureName></PrimaryAxis><SecondaryAxis><DefinedDirection>+X</DefinedDirection><Source>ReferenceFrame</Source><SourceDirection>-Z</SourceDirection><FeatureName></FeatureName></SecondaryAxis></Value></Frame><Frame><Id>Frame6</Id><Value><Name>F6</Name><Origin><Source>GeometricFeature</Source><FeatureName>circular curve 17</FeatureName></Origin><PrimaryAxis><DefinedDirection>+Y</DefinedDirection><Source>ReferenceFrame</Source><SourceDirection>+Y</SourceDirection><FeatureName></FeatureName></PrimaryAxis><SecondaryAxis><DefinedDirection>+X</DefinedDirection><Source>ReferenceFrame</Source><SourceDirection>-Z</SourceDirection><FeatureName></FeatureName></SecondaryAxis></Value></Frame></Frames>
  F1 : PMIOPort  Side=Left
  F2 : PMIOPort  Port=2  Side=Right
  G : PMIOPort  Port=3  Side=Left
  connections:
  frame_regular3/RConn1 -- F2/RConn1
  F1/RConn1 -- frame_regular3/LConn1
  File Solid3/RConn1 -- frame_regular3/LConn2
  frame_regular3/LConn4 -- G/RConn1
  File Solid1/RConn1 -- frame_regular3/LConn3
  File Solid4/RConn1 -- frame_regular3/RConn3
  File Solid2/RConn1 -- frame_regular3/RConn2

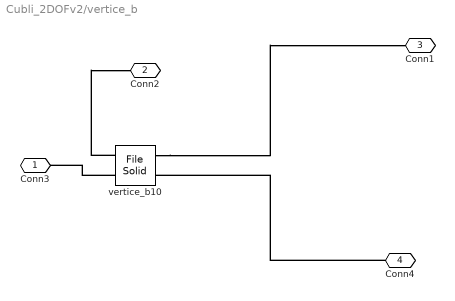
== system Cubli_2DOFv2/vertice_b ==
  vertice_b10 : sm_lib/Body Elements/File Solid  ExtGeomFileName=stp\bloque_vertice_b.STEP  UnitType=FromFile  ExtGeomFileUnits=m  StepReaderType=HEX  ExportConvexHullGeometry=off  InertiaType=CalculateFromGeometry  BasedOnType=Mass  Density=1000  DensityUnits=kg/m^3  Mass=2  MassUnits=g  CenterOfMass=[0 0 0]  CenterOfMassUnits=m  MomentsOfInertia=[1 1 1]  MomentsOfInertiaUnits=kg*m^2  ProductsOfInertia=[0 0 0]  ProductsOfInertiaUnits=kg*m^2  GraphicType=FromGeometry  MarkerShape=Sphere  MarkerSize=10  GraphicVisPropType=SimpleVisualProperties  GraphicDiffuseColor=[0.4392 1 0.1608]  GraphicOpacity=1  GraphicSpecularColor=[0.5 0.5 0.5 1.0]  GraphicAmbientColor=[0.15 0.15 0.15 1.0]  GraphicEmissiveColor=[0.0 0.0 0.0 1.0]  GraphicShininess=75  DoExposeReferenceFrame=off  SerializedFrames=<Frames><Frame><Id>Frame1</Id><Value><Name>F1</Name><Origin><Source>GeometricFeature</Source><FeatureName>planar surface 7</FeatureName></Origin><PrimaryAxis><DefinedDirection>+X</DefinedDirection><Source>ReferenceFrame</Source><SourceDirection>+Y</SourceDirection><FeatureName></FeatureName></PrimaryAxis><SecondaryAxis><DefinedDirection>+Y</DefinedDirection><Source>ReferenceFrame</Source><SourceDirection>-X</SourceDirection><FeatureName></FeatureName></SecondaryAxis></Value></Frame><Frame><Id>Frame2</Id><Value><Name>F2</Name><Origin><Source>GeometricFeature</Source><FeatureName>planar surface 10</FeatureName></Origin><PrimaryAxis><DefinedDirection>+X</DefinedDirection><Source>ReferenceFrame</Source><SourceDirection>-Z</SourceDirection><FeatureName></FeatureName></PrimaryAxis><SecondaryAxis><DefinedDirection>+Y</DefinedDirection><Source>ReferenceFrame</Source><SourceDirection>-Y</SourceDirection><FeatureName></FeatureName></SecondaryAxis></Value></Frame><Frame><Id>Frame3</Id><Value><Name>F3</Name><Origin><Source>GeometricFeature</Source><FeatureName>point 108</FeatureName></Origin><PrimaryAxis><DefinedDirection>+Z</DefinedDirection><Source>ReferenceFrame</Source><SourceDirection>+X</SourceDirection><FeatureName>segment 27</FeatureName></PrimaryAxis><SecondaryAxis><DefinedDirection>+X</DefinedDirection><Source>GeometricFeature</Source><SourceDirection>+X</SourceDirection><FeatureName>segment 37</FeatureName></SecondaryAxis></Value></Frame><Frame><Id>Frame4</Id><Value><Name>F4</Name><Origin><Source>GeometricFeature</Source><FeatureName>planar surface 13</FeatureName></Origin><PrimaryAxis><DefinedDirection>+Y</DefinedDirection><Source>ReferenceFrame</Source><SourceDirection>-Z</SourceDirection><FeatureName></FeatureName></PrimaryAxis><SecondaryAxis><DefinedDirection>+X</DefinedDirection><Source>ReferenceFrame</Source><SourceDirection>+X</SourceDirection><FeatureName></FeatureName></SecondaryAxis></Value></Frame></Frames>
  Conn3 : PMIOPort  Side=Left
  Conn2 : PMIOPort  Port=2  Side=Left
  Conn1 : PMIOPort  Port=3  Side=Right
  Conn4 : PMIOPort  Port=4  Side=Right
  connections:
  vertice_b10/LConn1 -- Conn2/RConn1
  Conn4/RConn1 -- vertice_b10/RConn2
  vertice_b10/RConn1 -- Conn1/RConn1
  vertice_b10/LConn2 -- Conn3/RConn1

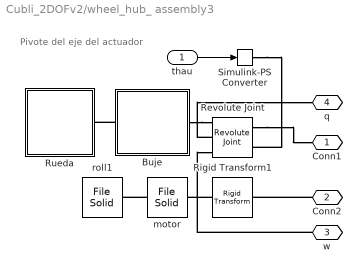
== system Cubli_2DOFv2/wheel_hub_ assembly3 ==
  note: Pivote del eje del actuador
  thau : Inport
  Buje : Subsystem
      mask Display: image('hub.jpg');
  Revolute Joint : sm_lib/Joints/Revolute Joint  JointMode=Normal  CompositeWrenchDir=FollowerOnBase  CompositeWrenchFrame=BaseFrame  SenseConstraintForce=off  SenseConstraintTorque=off  SenseTotalForce=off  SenseTotalTorque=off  PositionTargetSpecify=off  PositionTargetPriority=High  PositionTargetValue=0  PositionTargetValueUnits=deg  VelocityTargetSpecify=off  VelocityTargetPriority=High  VelocityTargetValue=0  VelocityTargetValueUnits=deg/s  EquilibriumPosition=0  EquilibriumPositionUnits=deg  SpringStiffness=0  SpringStiffnessUnits=N*m/deg  DampingCoefficient=Cw  DampingCoefficientUnits=N*m*s/rad  LowerLimitSpecify=off  LowerLimitBound=-90  LowerLimitBoundUnits=deg  LowerLimitStiffness=1e4  LowerLimitStiffnessUnits=N*m/deg  LowerLimitDamping=10  LowerLimitDampingUnits=N*m/(deg/s)  LowerLimitTransitionRegionWidth=0.1  LowerLimitTransitionRegionWidthUnits=deg  UpperLimitSpecify=off  UpperLimitBound=90  UpperLimitBoundUnits=deg  UpperLimitStiffness=1e4  UpperLimitStiffnessUnits=N*m/deg  UpperLimitDamping=10  UpperLimitDampingUnits=N*m/(deg/s)  UpperLimitTransitionRegionWidth=0.1  UpperLimitTransitionRegionWidthUnits=deg  TorqueActuationMode=InputTorque  MotionActuationMode=ComputedMotion  SensePosition=on  SenseVelocity=on  SenseAcceleration=off  SenseTorqueForce=off  SenseLowerLimitTorqueForce=off  SenseUpperLimitTorqueForce=off
  Rigid Transform1 : sm_lib/Frames and Transforms/Rigid Transform  RotationMethod=StandardAxis  FollAlignAxisA=+X  BaseAlignAxisA=+Y  FollAlignAxisB=+Y  BaseAlignAxisB=+Z  RotationStandardAxis=+X  RotationAngle=120  RotationAngleUnits=deg  RotationArbitraryAxis=[0 0 1]  RotationSequenceAxes=FollowerAxes  RotationSequence=XYX  RotationSequenceAngles=[0 0 0]  RotationSequenceAnglesUnits=deg  RotationMatrix=[1 0 0;0 1 0;0 0 1]  Quaternion=[1 0 0 0]  TranslationMethod=None  TranslationCartesianOffset=[0 0 0]  TranslationCartesianOffsetUnits=m  TranslationStandardAxis=+Z  TranslationStandardOffset=0  TranslationStandardOffsetUnits=m  TranslationROffset=0  TranslationROffsetUnits=m  TranslationThetaOffset=0  TranslationThetaOffsetUnits=deg  TranslationZOffset=0  TranslationZOffsetUnits=m
  Rueda : Subsystem
      mask Display: image('wheel.jpg');
  Simulink-PS Converter : nesl_utility/Simulink-PS Converter  PhysicalDomain=network_engine_domain  SubClassName=ps_input  LeftPortType=input  RightPortType=output  PseudoPeriodic=off  Frequencies=[]  NoiseDistribution=none  NoiseParameters=[]  Unit=N*m  AffineConversion=off  FilteringAndDerivatives=provide  SimscapeFilterOrder=1  InputFilterTimeConstant=0.001  UdotUserProvided=0
  motor : sm_lib/Body Elements/File Solid  ExtGeomFileName=stp\ECXFL42S KL A HTQ 24V_stp2.STEP  UnitType=FromFile  ExtGeomFileUnits=m  StepReaderType=HEX  ExportConvexHullGeometry=off  InertiaType=CalculateFromGeometry  BasedOnType=Mass  Density=1000  DensityUnits=kg/m^3  Mass=106  MassUnits=g  CenterOfMass=[0 0 0]  CenterOfMassUnits=m  MomentsOfInertia=[1 1 1]  MomentsOfInertiaUnits=kg*m^2  ProductsOfInertia=[0 0 0]  ProductsOfInertiaUnits=kg*m^2  GraphicType=FromGeometry  MarkerShape=Sphere  MarkerSize=10  GraphicVisPropType=SimpleVisualProperties  GraphicDiffuseColor=[0.149 0.149 0.149]  GraphicOpacity=1  GraphicSpecularColor=[0.5 0.5 0.5 1.0]  GraphicAmbientColor=[0.15 0.15 0.15 1.0]  GraphicEmissiveColor=[0.0 0.0 0.0 1.0]  GraphicShininess=75  DoExposeReferenceFrame=on  SerializedFrames=<Frames><Frame><Id>Frame1</Id><Value><Name>F1</Name><Origin><Source>GeometricFeature</Source><FeatureName>circular curve 413</FeatureName></Origin><PrimaryAxis><DefinedDirection>+Z</DefinedDirection><Source>ReferenceFrame</Source><SourceDirection>+Z</SourceDirection><FeatureName></FeatureName></PrimaryAxis><SecondaryAxis><DefinedDirection>+X</DefinedDirection><Source>ReferenceFrame</Source><SourceDirection>+X</SourceDirection><FeatureName></FeatureName></SecondaryAxis></Value></Frame></Frames>
  roll1 : sm_lib/Body Elements/File Solid  ExtGeomFileName=stp\instrument ball bearing_68_am.STEP  UnitType=FromFile  ExtGeomFileUnits=m  StepReaderType=HEX  ExportConvexHullGeometry=off  InertiaType=CalculateFromGeometry  BasedOnType=Mass  Density=1000  DensityUnits=kg/m^3  Mass=1.5  MassUnits=g  CenterOfMass=[0 0 0]  CenterOfMassUnits=m  MomentsOfInertia=[1 1 1]  MomentsOfInertiaUnits=kg*m^2  ProductsOfInertia=[0 0 0]  ProductsOfInertiaUnits=kg*m^2  GraphicType=FromGeometry  MarkerShape=Sphere  MarkerSize=10  GraphicVisPropType=SimpleVisualProperties  GraphicDiffuseColor=[0.5 0.5 0.5]  GraphicOpacity=1  GraphicSpecularColor=[0.5 0.5 0.5 1.0]  GraphicAmbientColor=[0.15 0.15 0.15 1.0]  GraphicEmissiveColor=[0.0 0.0 0.0 1.0]  GraphicShininess=75  DoExposeReferenceFrame=off  SerializedFrames=<Frames><Frame><Id>Frame1</Id><Value><Name>F1</Name><Origin><Source>GeometricFeature</Source><FeatureName>circular curve 23</FeatureName></Origin><PrimaryAxis><DefinedDirection>+Z</DefinedDirection><Source>ReferenceFrame</Source><SourceDirection>+Z</SourceDirection><FeatureName></FeatureName></PrimaryAxis><SecondaryAxis><DefinedDirection>+X</DefinedDirection><Source>ReferenceFrame</Source><SourceDirection>-X</SourceDirection><FeatureName></FeatureName></SecondaryAxis></Value></Frame></Frames>
  Conn1 : PMIOPort  Side=Left
  Conn2 : PMIOPort  Port=2  Side=Left
  w : PMIOPort  Port=3  Side=Right
  q : PMIOPort  Port=4  Side=Right
  wires:
  thau/1 -> Simulink-PS Converter/1
  connections:
  Conn2/RConn1 -- Rigid Transform1/LConn1
  Buje/RConn1 -- Revolute Joint/RConn1
  motor/LConn1 -- roll1/LConn1
  Revolute Joint/LConn1 -- Conn1/RConn1
  Rigid Transform1/RConn1 -- motor/RConn1
  Simulink-PS Converter/RConn1 -- Revolute Joint/LConn2
  Buje/LConn1 -- Rueda/RConn1
  w/RConn1 -- Revolute Joint/RConn3
  Revolute Joint/RConn2 -- q/RConn1
